simulink model "KociolBud3CvwCvg"  (R2026a)
settings: Solver=ode45  StopTime=6000  MaxStep=0.1  EnableMultiTasking=on
values from neighbouring files (symbols this model uses):
  cpw = 4200    [KociolBud_skryptWN.m]
  Cvk = cpw*row*Vk/skala    [KociolBud_skryptWN.m]
  czas_skok = 500    [KociolBud_Badania.m]
  dFg = [0, 0, 0] .* FgN    [KociolBud_Badania.m]
  dQd = [0, 0, 0] .* QgN    [KociolBud_Badania.m]
  dQk = 0.1*QkN    [KociolBud_Badania.m]
  dSP = 1    [KociolBud_Badania.m]
  dTzew = 0    [KociolBud_Badania.m]
  Fg0 = [1, 1, 1] .* FgN    [KociolBud_Badania.m]
  Ki_mp = 1/Ti_mp    (= 0.0030303030303)    [KociolBud_Badania.m]
  Kp_mp = 0.9/a_mp    [KociolBud_Badania.m]
  Qd0 = [0, 0, 0]    [KociolBud_Badania.m]
  Qk0 = QkN*1    [KociolBud_Badania.m]
  SP0 = Twew0(1)    [KociolBud_Badania.m]
  tau_siec = 240 / skala    [KociolBud_skryptWN.m]
  Tgp032 = (Tgp0(3)*Fg0(3) + Tgp0(2)*Fg0(2)  )   /   (  Fg0(3)+Fg0(2)    )    [KociolBud_skryptP0.m]
  Tgp0321 = (Tgp0(3)*Fg0(3) + Tgp0(2)*Fg0(2)  + Tgp0(1)*Fg0(1)  )   /   (  Fg0(3) + Fg0(2) + Fg0(1)    )    [KociolBud_skryptP0.m]
  Tkz0 = x0( IlePom*2+1)    [KociolBud_skryptP0.m]
  Tzew0 = TzewN    [KociolBud_Badania.m]
undefined symbols (not defined in the file or in its folder): Cvg, Cvw, Kcg, Kcw, Tgp0, Twew0
settings Model: Creator=Mateusz  LastModifiedBy=mmaks
settings DataIOCC: SignalLoggingSaveFormat=ModelDataLogs
settings DebuggingCC: UnderspecifiedInitializationDetection=Classic
settings HardwareCC: ProdHWDeviceType=32-bit Generic
settings GRTTargetCC: CombineOutputUpdateFcns=off  GRTInterface=on

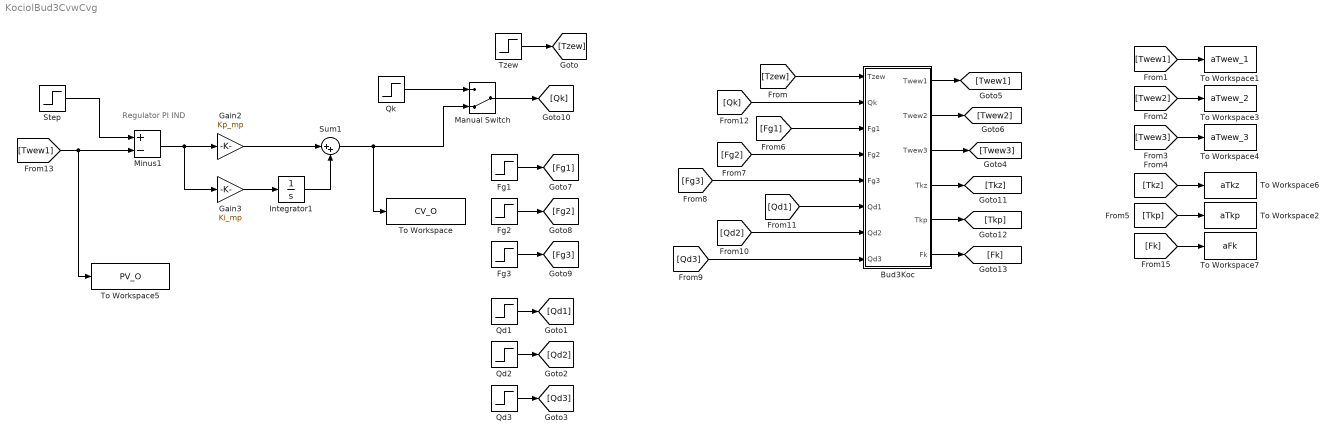
== system KociolBud3CvwCvg ==
  note: Regulator PI IND
  Bud3Koc : Subsystem
  Fg1 : Step  Time=czas_skok  InitialValue=Fg0(1)  FinalValue=Fg0(1)+dFg(1)  SampleTime=0
  Fg2 : Step  Time=czas_skok  InitialValue=Fg0(2)  FinalValue=Fg0(2)+dFg(2)  SampleTime=0
  Fg3 : Step  Time=czas_skok  InitialValue=Fg0(3)  FinalValue=Fg0(3)+dFg(3)  SampleTime=0
  Gain2 : Gain  Gain=Kp_mp
  Gain3 : Gain  Gain=Ki_mp
  Integrator1 : Integrator
  Manual Switch : ManualSwitch  CurrentSetting=0
  Minus1 : Sum  Inputs=+-
  Qd1 : Step  Time=czas_skok  InitialValue=Qd0(1)  FinalValue=Qd0(1)+dQd(1)  SampleTime=0
  Qd2 : Step  Time=czas_skok  InitialValue=Qd0(2)  FinalValue=Qd0(2)+dQd(2)  SampleTime=0
  Qd3 : Step  Time=czas_skok  InitialValue=Qd0(3)  FinalValue=Qd0(3)+dQd(3)  SampleTime=0
  Qk : Step  Time=czas_skok  InitialValue=Qk0  FinalValue=Qk0 + dQk  SampleTime=0
  Step : Step  Time=czas_skok  InitialValue=SP0  FinalValue=SP0 + dSP  SampleTime=0
  Sum1 : Sum  Inputs=|++
  To Workspace : ToWorkspace  VariableName=CV_O  SampleTime=-1
  To Workspace1 : ToWorkspace  VariableName=aTwew_1  SampleTime=-1
  To Workspace2 : ToWorkspace  VariableName=aTkp  SampleTime=-1
  To Workspace3 : ToWorkspace  VariableName=aTwew_2  SampleTime=-1
  To Workspace4 : ToWorkspace  VariableName=aTwew_3  SampleTime=-1
  To Workspace5 : ToWorkspace  VariableName=PV_O  SampleTime=-1
  To Workspace6 : ToWorkspace  VariableName=aTkz  SampleTime=-1
  To Workspace7 : ToWorkspace  VariableName=aFk  SampleTime=-1
  Tzew : Step  Time=czas_skok  InitialValue=Tzew0  FinalValue=Tzew0+dTzew  SampleTime=0
  wires:
  Tzew/1 -> [Tzew]
  Fg1/1 -> [Fg1]
  Fg2/1 -> [Fg2]
  Fg3/1 -> [Fg3]
  Bud3Koc/2(Twew2) -> [Twew2]
  [Tzew] -> Bud3Koc/1(Tzew)
  [Fg1] -> Bud3Koc/3(Fg1)
  [Fg2] -> Bud3Koc/4(Fg2)
  [Fg3] -> Bud3Koc/5(Fg3)
  Qd1/1 -> [Qd1]
  Qd2/1 -> [Qd2]
  Qd3/1 -> [Qd3]
  [Twew1] -> To Workspace1/1
  [Twew2] -> To Workspace3/1
  [Twew3] -> To Workspace4/1
  Bud3Koc/4(Tkz) -> [Tkz]
  Bud3Koc/5(Tkp) -> [Tkp]
  [Tkz] -> To Workspace6/1
  [Tkp] -> To Workspace2/1
  [Qd3] -> Bud3Koc/8(Qd3)
  [Qd2] -> Bud3Koc/7(Qd2)
  [Qd1] -> Bud3Koc/6(Qd1)
  Bud3Koc/6(Fk) -> [Fk]
  [Fk] -> To Workspace7/1
  Bud3Koc/3(Twew3) -> [Twew3]
  Minus1/1 -> Gain3/1, Gain2/1
  Integrator1/1 -> Sum1/2
  Sum1/1 -> Manual Switch/2, To Workspace/1
  Gain2/1 -> Sum1/1
  Gain3/1 -> Integrator1/1
  Bud3Koc/1(Twew1) -> [Twew1]
  Qk/1 -> Manual Switch/1
  [Qk] -> Bud3Koc/2(Qk)
  Manual Switch/1 -> [Qk]
  [Twew1] -> To Workspace5/1, Minus1/2
  Step/1 -> Minus1/1

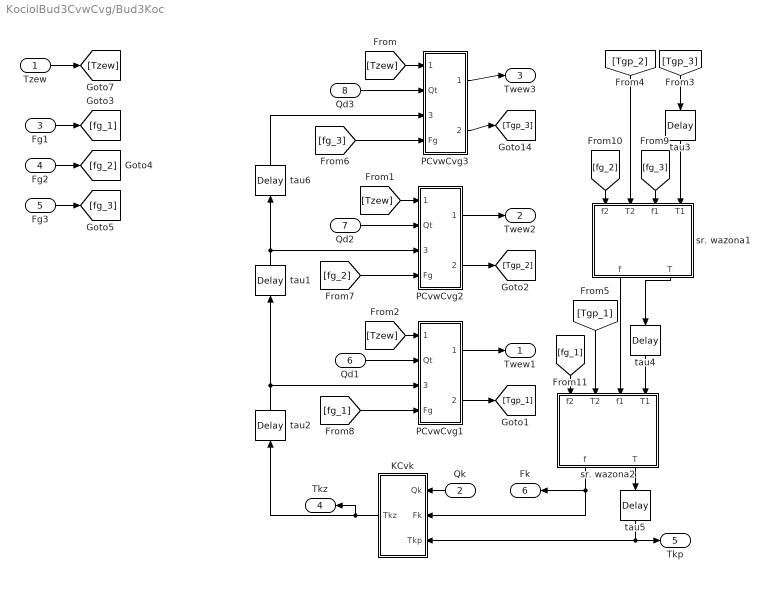
== system KociolBud3CvwCvg/Bud3Koc ==
  Tzew : Inport
  Qk : Inport  Port=2
  Fg1 : Inport  Port=3
  Fg2 : Inport  Port=4
  Fg3 : Inport  Port=5
  Qd1 : Inport  Port=6
  Qd2 : Inport  Port=7
  Qd3 : Inport  Port=8
  KCvk : Subsystem  mask{cpw=cpw, Cvk=Cvk, Tkz0=Tkz0}
  PCvwCvg1 : Subsystem  mask{cpw=cpw, Kcw=Kcw(1), Kcg=Kcg(1), Cvw=Cvw(1), Cvg=Cvg(1), Twew0=Twew0(1), Tgp0=Tgp0(1)}
  PCvwCvg2 : Subsystem  mask{cpw=cpw, Kcw=Kcw(2), Kcg=Kcg(2), Cvw=Cvw(2), Cvg=Cvg(2), Twew0=Twew0(2), Tgp0=Tgp0(2)}
  PCvwCvg3 : Subsystem  mask{cpw=cpw, Kcw=Kcw(3), Kcg=Kcg(3), Cvw=Cvw(3), Cvg=Cvg(3), Twew0=Twew0(3), Tgp0=Tgp0(3)}
  sr. wazona1 : Subsystem
  sr. wazona2 : Subsystem
  tau1 : TransportDelay  DelayTime=tau_siec  InitialOutput=Tkz0
  tau2 : TransportDelay  DelayTime=tau_siec  InitialOutput=Tkz0
  tau3 : TransportDelay  DelayTime=tau_siec  InitialOutput=Tgp0(3)
  tau4 : TransportDelay  DelayTime=tau_siec  InitialOutput=Tgp032
  tau5 : TransportDelay  DelayTime=tau_siec  InitialOutput=Tgp0321
  tau6 : TransportDelay  DelayTime=tau_siec  InitialOutput=Tkz0
  Twew1 : Outport
  Twew2 : Outport  Port=2
  Twew3 : Outport  Port=3
  Tkz : Outport  Port=4
  Tkp : Outport  Port=5
  Fk : Outport  Port=6
  wires:
  tau1/1 -> tau6/1, PCvwCvg2/3(Tgz)
  tau2/1 -> tau1/1, PCvwCvg1/3(Tgz)
  KCvk/1(Tkz) -> tau2/1, Tkz/1
  Qd2/1 -> PCvwCvg2/2(Qt)
  sr. wazona1/2(T) -> tau4/1
  tau3/1 -> sr. wazona1/4(T1)
  sr. wazona2/2(T) -> tau5/1
  tau5/1 -> Tkp/1, KCvk/3(Tkp)
  sr. wazona2/1(f) -> Fk/1, KCvk/2(Fk)
  tau4/1 -> sr. wazona2/4(T1)
  sr. wazona1/1(f) -> sr. wazona2/3(f1)
  [Tzew] -> PCvwCvg2/1(Tzew)
  PCvwCvg1/2(Tgp) -> [Tgp_1]
  PCvwCvg2/2(Tgp) -> [Tgp_2]
  [Tgp_3] -> tau3/1
  [Tgp_2] -> sr. wazona1/2(T2)
  [Tgp_1] -> sr. wazona2/2(T2)
  [fg_3] -> sr. wazona1/3(f1)
  [fg_2] -> sr. wazona1/1(f2)
  [fg_1] -> sr. wazona2/1(f2)
  Qk/1 -> KCvk/1(Qk)
  Tzew/1 -> [Tzew]
  PCvwCvg1/1(Twew) -> Twew1/1
  PCvwCvg2/1(Twew) -> Twew2/1
  Qd1/1 -> PCvwCvg1/2(Qt)
  [Tzew] -> PCvwCvg1/1(Tzew)
  PCvwCvg3/2(Tgp) -> [Tgp_3]
  PCvwCvg3/1(Twew) -> Twew3/1
  Qd3/1 -> PCvwCvg3/2(Qt)
  [Tzew] -> PCvwCvg3/1(Tzew)
  Fg1/1 -> [fg_1]
  Fg2/1 -> [fg_2]
  Fg3/1 -> [fg_3]
  [fg_3] -> PCvwCvg3/4(Fg)
  [fg_2] -> PCvwCvg2/4(Fg)
  [fg_1] -> PCvwCvg1/4(Fg)
  tau6/1 -> PCvwCvg3/3(Tgz)

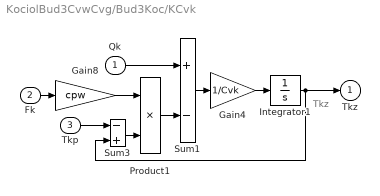
== system KociolBud3CvwCvg/Bud3Koc/KCvk ==
  note: Tkz
  Qk : Inport
  Fk : Inport  Port=2
  Tkp : Inport  Port=3
  Gain4 : Gain  Gain=1/Cvk  SaturateOnIntegerOverflow=on  OutDataTypeStr=Inherit: Same as input  ParamDataTypeStr=Inherit: Same as input
  Gain8 : Gain  Gain=cpw  SaturateOnIntegerOverflow=on  OutDataTypeStr=Inherit: Same as input  ParamDataTypeStr=Inherit: Same as input
  Integrator1 : Integrator  InitialCondition=Tkz0
  Product1 : Product  Inputs=**  InputSameDT=on  RndMeth=Zero  SaturateOnIntegerOverflow=on  OutDataTypeStr=Inherit: Same as first input
  Sum1 : Sum  Inputs=+-  InputSameDT=on  SaturateOnIntegerOverflow=on  OutDataTypeStr=Inherit: Same as first input
  Sum3 : Sum  Inputs=-+  InputSameDT=on  SaturateOnIntegerOverflow=on  OutDataTypeStr=Inherit: Same as first input
  Tkz : Outport
  wires:
  Fk/1 -> Gain8/1
  Sum3/1 -> Product1/2
  Gain8/1 -> Product1/1
  Qk/1 -> Sum1/1
  Gain4/1 -> Integrator1/1
  Sum1/1 -> Gain4/1
  Product1/1 -> Sum1/2
  Integrator1/1 -> Tkz/1, Sum3/2
  Tkp/1 -> Sum3/1

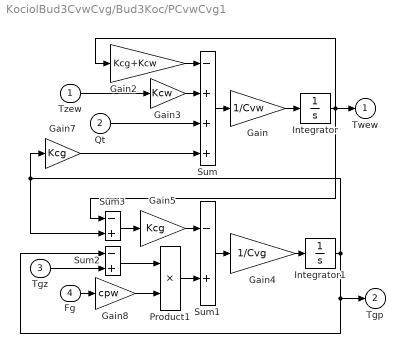
== system KociolBud3CvwCvg/Bud3Koc/PCvwCvg1 ==
  Tzew : Inport
  Qt : Inport  Port=2
  Tgz : Inport  Port=3
  Fg : Inport  Port=4
  Gain : Gain  Gain=1/Cvw  SaturateOnIntegerOverflow=on  OutDataTypeStr=Inherit: Same as input  ParamDataTypeStr=Inherit: Same as input
  Gain2 : Gain  Gain=Kcg+Kcw  SaturateOnIntegerOverflow=on  OutDataTypeStr=Inherit: Same as input  ParamDataTypeStr=Inherit: Same as input
  Gain3 : Gain  Gain=Kcw  SaturateOnIntegerOverflow=on  OutDataTypeStr=Inherit: Same as input  ParamDataTypeStr=Inherit: Same as input
  Gain4 : Gain  Gain=1/Cvg  SaturateOnIntegerOverflow=on  OutDataTypeStr=Inherit: Same as input  ParamDataTypeStr=Inherit: Same as input
  Gain5 : Gain  Gain=Kcg  SaturateOnIntegerOverflow=on  OutDataTypeStr=Inherit: Same as input  ParamDataTypeStr=Inherit: Same as input
  Gain7 : Gain  Gain=Kcg  SaturateOnIntegerOverflow=on  OutDataTypeStr=Inherit: Same as input  ParamDataTypeStr=Inherit: Same as input
  Gain8 : Gain  Gain=cpw  SaturateOnIntegerOverflow=on  OutDataTypeStr=Inherit: Same as input  ParamDataTypeStr=Inherit: Same as input
  Integrator : Integrator  InitialCondition=Twew0
  Integrator1 : Integrator  InitialCondition=Tgp0
  Product1 : Product  Inputs=**  InputSameDT=on  RndMeth=Zero  SaturateOnIntegerOverflow=on  OutDataTypeStr=Inherit: Same as first input
  Sum : Sum  Inputs=-+++  InputSameDT=on  SaturateOnIntegerOverflow=on  OutDataTypeStr=Inherit: Same as first input
  Sum1 : Sum  Inputs=-+  InputSameDT=on  SaturateOnIntegerOverflow=on  OutDataTypeStr=Inherit: Same as first input
  Sum2 : Sum  Inputs=-+  InputSameDT=on  SaturateOnIntegerOverflow=on  OutDataTypeStr=Inherit: Same as first input
  Sum3 : Sum  Inputs=-+  InputSameDT=on  SaturateOnIntegerOverflow=on  OutDataTypeStr=Inherit: Same as first input
  Twew : Outport
  Tgp : Outport  Port=2
  wires:
  Integrator/1 -> Sum3/1, Twew/1, Gain2/1
  Gain/1 -> Integrator/1
  Gain7/1 -> Sum/4
  Qt/1 -> Sum/3
  Tzew/1 -> Gain3/1
  Sum/1 -> Gain/1
  Gain3/1 -> Sum/2
  Gain2/1 -> Sum/1
  Fg/1 -> Gain8/1
  Gain4/1 -> Integrator1/1
  Sum1/1 -> Gain4/1
  Sum2/1 -> Product1/1
  Gain8/1 -> Product1/2
  Product1/1 -> Sum1/2
  Sum3/1 -> Gain5/1
  Gain5/1 -> Sum1/1
  Integrator1/1 -> Tgp/1, Sum2/1, Gain7/1, Sum3/2
  Tgz/1 -> Sum2/2

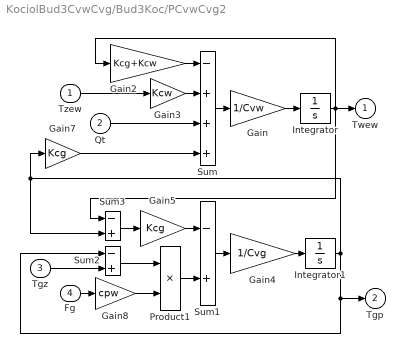
== system KociolBud3CvwCvg/Bud3Koc/PCvwCvg2 ==
  Tzew : Inport
  Qt : Inport  Port=2
  Tgz : Inport  Port=3
  Fg : Inport  Port=4
  Gain : Gain  Gain=1/Cvw  SaturateOnIntegerOverflow=on  OutDataTypeStr=Inherit: Same as input  ParamDataTypeStr=Inherit: Same as input
  Gain2 : Gain  Gain=Kcg+Kcw  SaturateOnIntegerOverflow=on  OutDataTypeStr=Inherit: Same as input  ParamDataTypeStr=Inherit: Same as input
  Gain3 : Gain  Gain=Kcw  SaturateOnIntegerOverflow=on  OutDataTypeStr=Inherit: Same as input  ParamDataTypeStr=Inherit: Same as input
  Gain4 : Gain  Gain=1/Cvg  SaturateOnIntegerOverflow=on  OutDataTypeStr=Inherit: Same as input  ParamDataTypeStr=Inherit: Same as input
  Gain5 : Gain  Gain=Kcg  SaturateOnIntegerOverflow=on  OutDataTypeStr=Inherit: Same as input  ParamDataTypeStr=Inherit: Same as input
  Gain7 : Gain  Gain=Kcg  SaturateOnIntegerOverflow=on  OutDataTypeStr=Inherit: Same as input  ParamDataTypeStr=Inherit: Same as input
  Gain8 : Gain  Gain=cpw  SaturateOnIntegerOverflow=on  OutDataTypeStr=Inherit: Same as input  ParamDataTypeStr=Inherit: Same as input
  Integrator : Integrator  InitialCondition=Twew0
  Integrator1 : Integrator  InitialCondition=Tgp0
  Product1 : Product  Inputs=**  InputSameDT=on  RndMeth=Zero  SaturateOnIntegerOverflow=on  OutDataTypeStr=Inherit: Same as first input
  Sum : Sum  Inputs=-+++  InputSameDT=on  SaturateOnIntegerOverflow=on  OutDataTypeStr=Inherit: Same as first input
  Sum1 : Sum  Inputs=-+  InputSameDT=on  SaturateOnIntegerOverflow=on  OutDataTypeStr=Inherit: Same as first input
  Sum2 : Sum  Inputs=-+  InputSameDT=on  SaturateOnIntegerOverflow=on  OutDataTypeStr=Inherit: Same as first input
  Sum3 : Sum  Inputs=-+  InputSameDT=on  SaturateOnIntegerOverflow=on  OutDataTypeStr=Inherit: Same as first input
  Twew : Outport
  Tgp : Outport  Port=2
  wires:
  Integrator/1 -> Sum3/1, Twew/1, Gain2/1
  Gain/1 -> Integrator/1
  Gain7/1 -> Sum/4
  Qt/1 -> Sum/3
  Tzew/1 -> Gain3/1
  Sum/1 -> Gain/1
  Gain3/1 -> Sum/2
  Gain2/1 -> Sum/1
  Fg/1 -> Gain8/1
  Gain4/1 -> Integrator1/1
  Sum1/1 -> Gain4/1
  Sum2/1 -> Product1/1
  Gain8/1 -> Product1/2
  Product1/1 -> Sum1/2
  Sum3/1 -> Gain5/1
  Gain5/1 -> Sum1/1
  Integrator1/1 -> Tgp/1, Sum2/1, Gain7/1, Sum3/2
  Tgz/1 -> Sum2/2

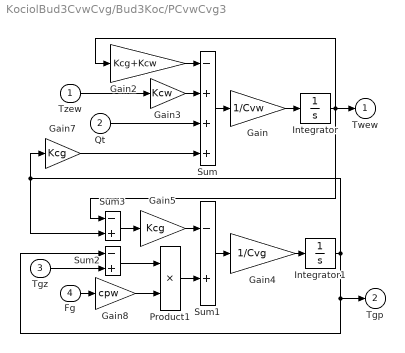
== system KociolBud3CvwCvg/Bud3Koc/PCvwCvg3 ==
  Tzew : Inport
  Qt : Inport  Port=2
  Tgz : Inport  Port=3
  Fg : Inport  Port=4
  Gain : Gain  Gain=1/Cvw  SaturateOnIntegerOverflow=on  OutDataTypeStr=Inherit: Same as input  ParamDataTypeStr=Inherit: Same as input
  Gain2 : Gain  Gain=Kcg+Kcw  SaturateOnIntegerOverflow=on  OutDataTypeStr=Inherit: Same as input  ParamDataTypeStr=Inherit: Same as input
  Gain3 : Gain  Gain=Kcw  SaturateOnIntegerOverflow=on  OutDataTypeStr=Inherit: Same as input  ParamDataTypeStr=Inherit: Same as input
  Gain4 : Gain  Gain=1/Cvg  SaturateOnIntegerOverflow=on  OutDataTypeStr=Inherit: Same as input  ParamDataTypeStr=Inherit: Same as input
  Gain5 : Gain  Gain=Kcg  SaturateOnIntegerOverflow=on  OutDataTypeStr=Inherit: Same as input  ParamDataTypeStr=Inherit: Same as input
  Gain7 : Gain  Gain=Kcg  SaturateOnIntegerOverflow=on  OutDataTypeStr=Inherit: Same as input  ParamDataTypeStr=Inherit: Same as input
  Gain8 : Gain  Gain=cpw  SaturateOnIntegerOverflow=on  OutDataTypeStr=Inherit: Same as input  ParamDataTypeStr=Inherit: Same as input
  Integrator : Integrator  InitialCondition=Twew0
  Integrator1 : Integrator  InitialCondition=Tgp0
  Product1 : Product  Inputs=**  InputSameDT=on  RndMeth=Zero  SaturateOnIntegerOverflow=on  OutDataTypeStr=Inherit: Same as first input
  Sum : Sum  Inputs=-+++  InputSameDT=on  SaturateOnIntegerOverflow=on  OutDataTypeStr=Inherit: Same as first input
  Sum1 : Sum  Inputs=-+  InputSameDT=on  SaturateOnIntegerOverflow=on  OutDataTypeStr=Inherit: Same as first input
  Sum2 : Sum  Inputs=-+  InputSameDT=on  SaturateOnIntegerOverflow=on  OutDataTypeStr=Inherit: Same as first input
  Sum3 : Sum  Inputs=-+  InputSameDT=on  SaturateOnIntegerOverflow=on  OutDataTypeStr=Inherit: Same as first input
  Twew : Outport
  Tgp : Outport  Port=2
  wires:
  Integrator/1 -> Sum3/1, Twew/1, Gain2/1
  Gain/1 -> Integrator/1
  Gain7/1 -> Sum/4
  Qt/1 -> Sum/3
  Tzew/1 -> Gain3/1
  Sum/1 -> Gain/1
  Gain3/1 -> Sum/2
  Gain2/1 -> Sum/1
  Fg/1 -> Gain8/1
  Gain4/1 -> Integrator1/1
  Sum1/1 -> Gain4/1
  Sum2/1 -> Product1/1
  Gain8/1 -> Product1/2
  Product1/1 -> Sum1/2
  Sum3/1 -> Gain5/1
  Gain5/1 -> Sum1/1
  Integrator1/1 -> Tgp/1, Sum2/1, Gain7/1, Sum3/2
  Tgz/1 -> Sum2/2

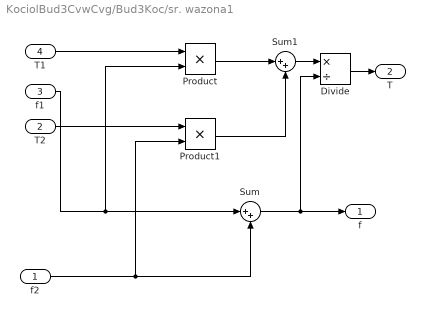
== system KociolBud3CvwCvg/Bud3Koc/sr. wazona1 ==
  f2 : Inport
  T2 : Inport  Port=2
  f1 : Inport  Port=3
  T1 : Inport  Port=4
  Divide : Product  Inputs=*/
  Product : Product  RndMeth=Zero
  Product1 : Product  RndMeth=Zero
  Sum : Sum  Inputs=|++
  Sum1 : Sum  Inputs=|++
  f : Outport
  T : Outport  Port=2
  wires:
  T1/1 -> Product/1
  T2/1 -> Product1/1
  f1/1 -> Product/2, Sum/1
  f2/1 -> Product1/2, Sum/2
  Product/1 -> Sum1/1
  Product1/1 -> Sum1/2
  Sum/1 -> f/1, Divide/2
  Sum1/1 -> Divide/1
  Divide/1 -> T/1

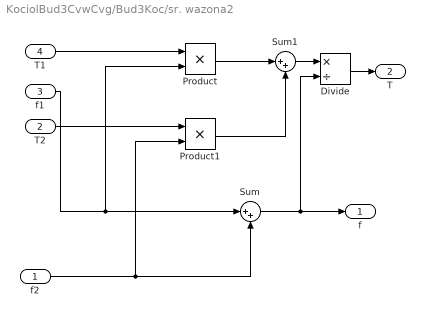
== system KociolBud3CvwCvg/Bud3Koc/sr. wazona2 ==
  f2 : Inport
  T2 : Inport  Port=2
  f1 : Inport  Port=3
  T1 : Inport  Port=4
  Divide : Product  Inputs=*/
  Product : Product  RndMeth=Zero
  Product1 : Product  RndMeth=Zero
  Sum : Sum  Inputs=|++
  Sum1 : Sum  Inputs=|++
  f : Outport
  T : Outport  Port=2
  wires:
  T1/1 -> Product/1
  T2/1 -> Product1/1
  f1/1 -> Product/2, Sum/1
  f2/1 -> Product1/2, Sum/2
  Product/1 -> Sum1/1
  Product1/1 -> Sum1/2
  Sum/1 -> f/1, Divide/2
  Sum1/1 -> Divide/1
  Divide/1 -> T/1
